simulink model "printable_simulation"  (R2024b)
settings: Solver=ode1be  StartTime=0.0  StopTime=10  FixedStep=0.001  RelTol=1e-3
model workspace (MAT data in the model file):
  AMP = 1
  FREQ = 1
  i_abc = 1
undefined symbols (not defined in the file or in its folder): Drive_wheel, Driveshaft, eff_shaft, f_OVD, i, J_S21, Jr2, K, M_curve_1, M_curve_2, M_total, mi_c, mi_s, Mode, N_clutch, n_curve_1, n_curve_2, n_max_1, n_max_2, n_surfaces, Pl, r_eq_clutch, r_geom, Shaft, sigma0, sigma1, sigma2, Spurs_Inertia, Stage1, Stage2, Stage3, vs, wheel_width
libraries: simulink x12, slpidlib x1
(part 1 of 3)
settings Model: Creator=menda  LastModifiedBy=menda
settings SolverCC: ZeroCrossAlgorithm=Adaptive
settings DebuggingCC: AlgebraicLoopMsg=none  IgnoredZcDiagnostic=none

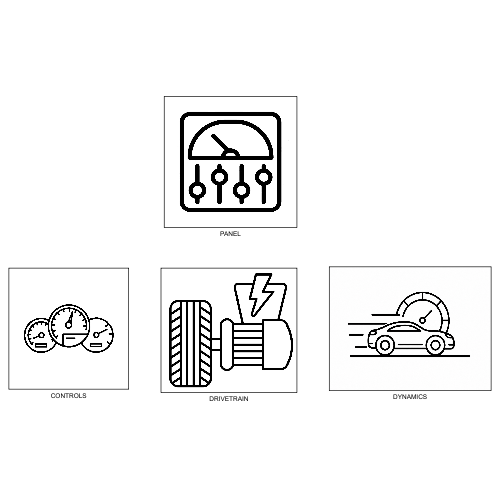
[thumbnail: Simulink's stored preview of the top-level diagram]
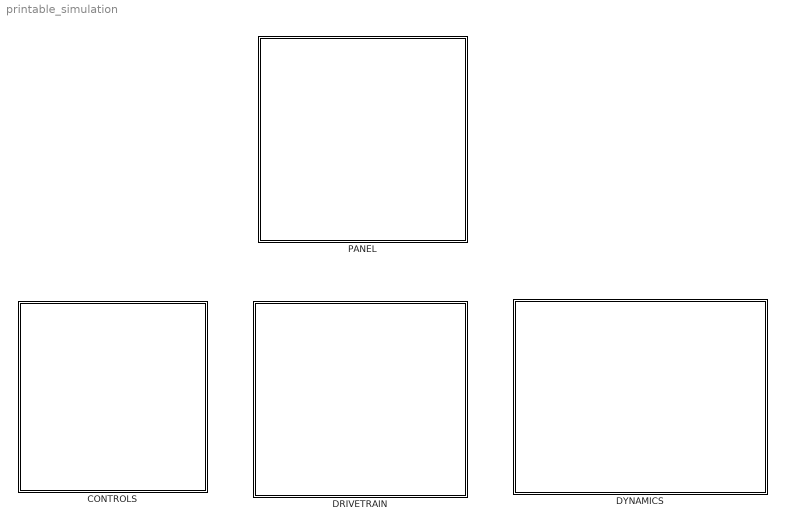
== system printable_simulation ==
  CONTROLS : Subsystem
      mask Display: image('images/controls.jpg');
  DRIVETRAIN : Subsystem
      mask Display: image('images/drivetrain_icon.png');
  DYNAMICS : Subsystem
      mask Display: image('images/Dynamics.png');
  PANEL : Subsystem
      mask Display: image('images/panel.jpg');

== system printable_simulation/CONTROLS ==
  MCU : Subsystem
      mask Display: image('images/MCU.jpg');
  Speed Profile : Subsystem
      mask Display: image('images/speedProfile.png');
  Speed control : Subsystem
      mask Display: image('images/speedControl.jpg');
  tag scope: Gear=global, M_Driver=global, M_MCU=global
  wires:
  Speed Profile/1(Target) -> Speed control/2(Target)  "v/a"
  Speed control/1(M_request) -> MCU/1(In1), [M_Driver]
  [Speed] -> Speed control/1(V_fdbk)
  MCU/1(Out1) -> [M_MCU]  "Torque"
  MCU/2(Out2) -> [Gear]  "Gear"

== system printable_simulation/DRIVETRAIN ==
  Motor : Subsystem
      mask Display: image("images/engine.jpg")
  Transmission : Subsystem
      mask Display: image('images/transmission.jpg');
  Wheel Model : Subsystem
      mask Display: image('images/wheel_model.jpg');
  Zero : Constant  Value=0  OutDataTypeStr=Inherit: Inherit via back propagation
  tag scope: F_wheel=global, M_engine=global
  wires:
  Motor/1(M_motor) -> Transmission/1(M_engine), [M_engine]
  Wheel Model/1("  ") -> [F_wheel]  "F_wheels"
  [M_MCU] -> Motor/1(M_MCU)
  Zero/1 -> Wheel Model/3(M_break)
  Transmission/1(M_tra) -> Wheel Model/2(M_tra)
  [V_load] -> Wheel Model/1(Vload)

== system printable_simulation/DYNAMICS ==
  Aerodynamic Forces : Subsystem
      mask Display: image('images/aerodynamic.png');
  Inclination : Subsystem
      mask Display: image('images/slope.jpg');
  Load Transfer : Subsystem
      mask Display: image('images/Load_transfer.png');
  Rolling Resistance : Subsystem
      mask Display: image('images/rolling_resistance.png');
  Sum : Sum  Inputs=-+-
  Vehicle Dynamics : Subsystem
      mask Display: image('images/Dynamics.png');
  tag scope: Speed=global, V_load=global
  wires:
  Sum/1 -> Vehicle Dynamics/1(Ft)
  Rolling Resistance/1(F) -> Sum/2  "F_T"
  Inclination/1(F_G) -> Sum/3  "F_G"
  Aerodynamic Forces/1(Fa) -> Sum/1  "D_A"
  Vehicle Dynamics/1(v) -> [Speed]  "v"
  [Speed] -> Rolling Resistance/1(v_x), Aerodynamic Forces/1(v_x)
  Load Transfer/1(Fz) -> [V_load]
  Vehicle Dynamics/2(acc) -> Load Transfer/1(acc)  "acc"
  Inclination/2(theta) -> Load Transfer/2(theta)  "theta"
  [F_wheel] -> Rolling Resistance/2(Fw)  "Fx"
  [V_load] -> Rolling Resistance/3(Fz)

== system printable_simulation/PANEL ==
  Differential and Driveshafts : Subsystem
      mask Display: image('images/transmission.jpg');
  Gearbox : Subsystem  Variant=on
      settings: PortSchema="{\"entries\":[{\"content\":{\"sides\":[{\"content\":{\"connectorIds\":[\"In1\"]},\"type\":\"ConnectorPlacement.EquallySpacedRectSide\",\"uuid\":\"205e71ba-e400-46cb-8798-7dc05ab83482\"},{\"content\":{\"connectorIds\":[\"Out1\"],\"side\":\"RIGHT\"},\"type\":\"ConnectorPlacement.EquallySpacedRectSide\",\"uuid\":\"765c3a3a-64c2-415f-a9cc-3b16fa892d5b\"},{\"content\":{\"connectorIds\":[\"In2\"],\"side\":\"TOP\"},\"type\":\"ConnectorPlacement.EquallySpacedRectSide\",\"uuid\":\"cfd783c5-1c77-446c-8167-ee8726316dc7\"}]},\"type\":\"ConnectorPlacement.EquallySpacedConnector\",\"uuid\":\"e0fc6072-49b0-4dfc-b677-eb2d55a08206\"}],\"packageUris\":[\"http://schema.mathworks.com/mf0/Connector/R2020b\"],\"version\":\"1.0\"}"
      mask Display: image('images/Gearbox.png');
  Main Control Unit : Subsystem
      settings: PortSchema="{\"entries\":[{\"content\":{\"sides\":[{\"content\":{\"connectorIds\":[\"In1\"]},\"type\":\"ConnectorPlacement.EquallySpacedRectSide\",\"uuid\":\"5eb0ff4b-93e1-4f3c-b7be-4fa0816a4baa\"},{\"content\":{\"side\":\"RIGHT\"},\"type\":\"ConnectorPlacement.EquallySpacedRectSide\",\"uuid\":\"5fe0ae6b-cde3-4045-ae61-047bb7dc3994\"},{\"content\":{\"side\":\"TOP\"},\"type\":\"ConnectorPlacement.EquallySpacedRectSide\",\"uuid\":\"de997b44-717c-495a-94b2-5a947ffcf83c\"},{\"content\":{\"connectorIds\":[\"Out1\",\"Out2\"],\"side\":\"BOTTOM\"},\"type\":\"ConnectorPlacement.EquallySpacedRectSide\",\"uuid\":\"4ff163e0-fe89-465b-a414-8c0cdfc889e5\"}]},\"type\":\"ConnectorPlacement.EquallySpacedConnector\",\"uuid\":\"bd974712-b545-4b72-b6b5-729f52311d40\"}],\"packageUris\":[\"http://schema.mathworks.com/mf0/Connector/R2020b\"],\"version\":\"1.0\"}"
      mask Display: image('images/MCU.jpg');
  Motor : Subsystem
      settings: PortSchema="{\"entries\":[{\"content\":{\"sides\":[{\"content\":{},\"type\":\"ConnectorPlacement.EquallySpacedRectSide\",\"uuid\":\"c3efcd4e-0739-476f-ba2f-028379b282a4\"},{\"content\":{\"connectorIds\":[\"Out1\"],\"side\":\"RIGHT\"},\"type\":\"ConnectorPlacement.EquallySpacedRectSide\",\"uuid\":\"1e8de8b1-ce2e-4e7d-9395-8c2bdb446185\"},{\"content\":{\"connectorIds\":[\"In1\"],\"side\":\"TOP\"},\"type\":\"ConnectorPlacement.EquallySpacedRectSide\",\"uuid\":\"8aefb245-65c2-4998-a20e-c273ac432bb8\"}]},\"type\":\"ConnectorPlacement.EquallySpacedConnector\",\"uuid\":\"e54aecd9-b953-4a93-9e93-d889ce431bd3\"}],\"packageUris\":[\"http://schema.mathworks.com/mf0/Connector/R2020b\"],\"version\":\"1.0\"}"
      mask Display: image("images/engine2.jpg")
  tag scope: M_tra=global
  wires:
  Motor/1(Out1) -> Gearbox/1(M_engine)  "M_motor"
  Main Control Unit/1(Out2) -> Motor/1(In1)  "M_MCU"
  Main Control Unit/2(Out1) -> Gearbox/2(Gear)  "Gear"
  Differential and Driveshafts/1(Out1) -> [M_tra]
  [M_Driver] -> Main Control Unit/1(In1)
  Gearbox/1(M_Diff) -> Differential and Driveshafts/1(In1)  "M_Diff"

== system printable_simulation/CONTROLS/MCU ==
  In1 : Inport
  clutchSet : Inport  Port=2
  AMT : Stateflow chart  Commented=on  TreatAsAtomicUnit=on
  Bus Creator : BusCreator  Inputs=2
  DCT_MCU : Stateflow chart  TreatAsAtomicUnit=on
      settings: PortSchema="{\"entries\":[{\"content\":{\"sides\":[{\"content\":{\"connectorIds\":[\"In2\",\"In1\",\"In14\",\"In9\",\"In4\",\"In5\",\"In6\",\"In16\",\"In8\",\"In15\",\"In11\",\"In12\",\"In10\",\"In13\",\"In7\",\"In3\",\"In17\"]},\"type\":\"ConnectorPlacement.EquallySpacedRectSide\",\"uuid\":\"1fb08156-1d34-4e57-90fe-6c8713929a60\"},{\"content\":{\"connectorIds\":[\"Out1\",\"Out2\",\"Out7\",\"Out4\",\"Out8\",\"Out9\",\"Out5\",\"Out6\",\"Out3\"],\"side\":\"RIGHT\"},\"type\":\"ConnectorPlacement.EquallySpacedRectSide\",\"uuid\":\"168ad19e-6ddc-4b37-b106-ff21161f873d\"},{\"content\":{\"side\":\"TOP\"},\"type\":\"ConnectorPlacement.EquallySpacedRectSide\",\"uuid\":\"0fbd732c-56c3-431e-92eb-9e0a9524aa51\"}]},\"type\":\"ConnectorPlacement.EquallySpacedConnector\",\"uuid\":\"e654060b-9493-42bd-b3b5-2b9fb4d828c1\"}],\"packageUris\":[\"http://schema.mathworks.com/mf0/Connector/R2020b\"],\"version\":\"1.0\"}"
  Gain : Gain
  Subsystem : Subsystem
  TDT : Stateflow chart  TreatAsAtomicUnit=on
  Out1 : Outport
  Out2 : Outport  Port=2
  C2 : Outport  Port=3
  tag scope: clutch=global, shifting_stage=global
  wires:
  In1/1 -> [shifting_stage], Bus Creator/1, Gain/1  "M_MCU1"
  Bus Creator/1 -> Out1/1
  Gain/1 -> Bus Creator/2  "M_MCU2"
  clutchSet/1 -> Subsystem/1(clutchSet)
  Subsystem/1(clutch) -> [clutch], C2/1

== system printable_simulation/CONTROLS/Speed Profile ==
  Acceleration Mode : Subsystem
      mask Display: image("images\AccProfile.jpg")
  Constant : Constant  Value=Mode
  Multiport Switch : MultiPortSwitch  SaturateOnIntegerOverflow=off  InputSameDT=off
  "Pedal Profile " : Subsystem
      mask Display: image("images/Pedal.jpg")
  WLTP Profile : Subsystem
      mask Display: image("images\WLTPprofile.png")
  Target : Outport
  wires:
  Multiport Switch/1 -> Target/1
  Acceleration Mode/1(Out1) -> Multiport Switch/2
  WLTP Profile/1(Out1) -> Multiport Switch/3
  "Pedal Profile "/1(Out1) -> Multiport Switch/4
  Constant/1 -> Multiport Switch/1

== system printable_simulation/CONTROLS/Speed control ==
  V_fdbk : Inport
  Target : Inport  Port=2
  Add : Sum  Inputs=+-
  Constant : Constant  Value=Mode
  Gain : Gain  Gain=3.6
  Gain1 : Gain  Gain=M_total
  Pedal Value Limiter : Saturate  UpperLimit=1  LowerLimit=-1
  Speed Control : slpidlib/PID Controller  Controller=PID  Form=Parallel  TimeDomain=Continuous-time  UseExternalTs=off  SampleTime=-1  IntegratorMethod=Forward Euler  FilterMethod=Forward Euler  ControllerParametersSource=internal  P=0.8  I=0.001  UseKiTs=off  D=0  UseExternalDerivativeSource=off  N=100  UseFilter=on  TunerSelectOption=Transfer Function Based (PID Tuner App)  InitialConditionSource=internal  InitialConditionForIntegrator=0  InitialConditionForFilter=0  DifferentiatorICPrevScaledInput=0  ExternalReset=none  TrackingMode=off  Kt=1  LimitOutput=off  SatLimitsSource=internal  UpperSaturationLimit=inf  LowerSaturationLimit=-inf  LinearizeAsGain=on  AntiWindupMode=none  Kb=1  LimitIntegrator=off  UpperIntegratorSaturationLimit=inf  LowerIntegratorSaturationLimit=-inf  POutMin=[]  POutMax=[]  IOutMin=[]  IOutMax=[]  DOutMin=[]  DOutMax=[]  NOutMin=[]  NOutMax=[]  SumOutMin=[]  SumOutMax=[]  SaturationOutMin=[]  SaturationOutMax=[]  PParamMin=[]  PParamMax=[]  IParamMin=[]  IParamMax=[]  DParamMin=[]  DParamMax=[]  NParamMin=[]  NParamMax=[]  KbParamMin=[]  KbParamMax=[]  KtParamMin=[]  KtParamMax=[]  KbOutMin=[]  KbOutMax=[]  KtOutMin=[]  KtOutMax=[]  IntegratorOutMin=[]  IntegratorOutMax=[]  FilterOutMin=[]  FilterOutMax=[]  SumI1OutMin=[]  SumI1OutMax=[]  SumI2OutMin=[]  SumI2OutMax=[]  SumI3OutMin=[]  SumI3OutMax=[]  SumI4OutMin=[]  SumI4OutMax=[]  SumDOutMin=[]  SumDOutMax=[]  DifferentiatorOutMin=[]  DifferentiatorOutMax=[]  FilterDiffOutCoefMin=[]  FilterDiffOutCoefMax=[]  ReciprocalOutMin=[]  ReciprocalOutMax=[]  SumDenOutMin=[]  SumDenOutMax=[]  SumNumOutMin=[]  SumNumOutMax=[]  DivideOutMin=[]  DivideOutMax=[]  UdiffTsProdOutMin=[]  UdiffTsProdOutMax=[]  NTsProdOutMin=[]  NTsProdOutMax=[]  UintegralTsProdOutMin=[]  UintegralTsProdOutMax=[]  UngainTsProdOutMin=[]  UngainTsProdOutMax=[]  ClampingZeroOutDataTypeStr=Inherit: Inherit via back propagation  ClampingZeroOutMin=[]  ClampingZeroOutMax=[]  FilterDenConstantOutDataTypeStr=Inherit: Inherit via back propagation  FilterDenConstantOutMin=[]  FilterDenConstantOutMax=[]  PCopyOutDataTypeStr=Inherit: Inherit via back propagation  PCopyOutMin=[]  PCopyOutMax=[]  NCopyOutDataTypeStr=Inherit: Inherit via back propagation  NCopyOutMin=[]  NCopyOutMax=[]  IntegratorContinuousStateAttributes=''  IntegratorStateMustResolveToSignalObject=off  IntegratorRTWStateStorageClass=Auto  FilterContinuousStateAttributes=''  FilterStateMustResolveToSignalObject=off  FilterRTWStateStorageClass=Auto  ParallelPVariant=InternalParameters  IdealPVariant=Disabled  IVariant=InternalParameters  DVariant=InternalParameters  IntegratorVariant=Continuous  SatVariant=Disabled  AWVariant=Passthrough  PCopyVariant=Disabled  TRVariant=Disabled  FdbkBlocksVariant=Forward  IdealPFdbkVariant=Disabled  SatFdbkVariant=Disabled  DerivativeFilterVariant=ContFilter  NVariant=InternalParameters  NCopyVariant=Disabled  FilterICVariant=InternalICsFilter  IntegratorICVariant=InternalICs  ExternalResetVariant=Disabled  TRSumVariant=Passthrough  SumFdbkVariant=Disabled  SumVariant=Sum_PID  TsampFilterVariant=InternalTs  TsampNgainVariant=Passthrough  TsampIntegralVariant=Disabled_SignalSpec  ExternalSaturationOutDataTypeStr=Inherit: Same as second input  DerivativeSourceVariant=ErrorSignal  PreIntVariant=InternalPreInt
  Switch : Switch  Criteria=u2 > Threshold  Threshold=2  SaturateOnIntegerOverflow=off  InputSameDT=off
  Transfer Fcn : TransferFcn  Denominator=[0.008 1]
  M_request : Outport
  tag scope: Pedal=global
  wires:
  Add/1 -> Speed Control/1  "v_error"
  Transfer Fcn/1 -> Gain1/1, [Pedal]  "Pedal_value"
  Constant/1 -> Switch/2
  Gain1/1 -> M_request/1
  Pedal Value Limiter/1 -> Switch/3
  Speed Control/1 -> Pedal Value Limiter/1
  Gain/1 -> Add/2
  Switch/1 -> Transfer Fcn/1
  Target/1 -> Add/1, Switch/1
  V_fdbk/1 -> Gain/1

== system printable_simulation/DRIVETRAIN/Motor ==
  M_MCU : Inport
  AND : Logic  Inputs=3  IconShape=distinctive  AllPortsSameDT=off  OutDataTypeStr=boolean
  Subsystem : Subsystem  Commented=on
  Subsystem1 : Subsystem  Commented=on
  Subsystem2 : Subsystem
  M_motor : Outport
  wires:
  M_MCU/1 -> Subsystem2/1(M_MCU), Subsystem1/1(M_MCU), Subsystem/1(M_MCU)
  Subsystem/1(M_motor) -> AND/3  "M_motor"
  AND/1 -> M_motor/1
  Subsystem1/1(M_motor) -> AND/2
  Subsystem2/1(M_motor) -> AND/1

== system printable_simulation/DRIVETRAIN/Transmission ==
  M_engine : Inport
  Differential and Driveshafts : Subsystem
      mask Display: image('images/transmission.jpg');
  Gearbox : Subsystem  Variant=on
      mask Display: image('images/branco.png');
  eff_GB : Gain  Gain=0.97
  M_tra : Outport
  wires:
  M_engine/1 -> Gearbox/1(M_motor)
  Gearbox/1(M_Diff) -> eff_GB/1
  eff_GB/1 -> Differential and Driveshafts/1(M_Diff)
  Differential and Driveshafts/1(M_shaftL) -> M_tra/1

== system printable_simulation/DRIVETRAIN/Wheel Model ==
  Vload : Inport
  M_tra : Inport  Port=2
  M_break : Inport  Port=3
  Front Wheels : Subsystem
      mask Display: image('images/branco.png');
  Product : Product
  Rear Wheels : Subsystem
      mask Display: image('images/branco.png');
  Sum : Sum  Inputs=+|+
  "  " : Outport
  tag scope: w_fdbk_tire=global
  wires:
  Sum/1 -> "  "/1
  Vload/1 -> Front Wheels/1(Vload), Rear Wheels/3(Vload)
  Rear Wheels/1(F_rear_wheels) -> Sum/1  "F_rear"
  Front Wheels/1(F_front_wheels) -> Sum/2  "F_front"
  M_tra/1 -> Rear Wheels/1(M_tra), Front Wheels/2(M_tra)
  M_break/1 -> Front Wheels/3(M_break), Rear Wheels/2(M_break)
  [Speed] -> Product/1
  [r_dyn] -> Product/2
  Product/1 -> [w_fdbk_tire]

== system printable_simulation/DYNAMICS/Aerodynamic Forces ==
  v_x : Inport
  Fa : Outport  VectorParamsAs1DForOutWhenUnconnected=off
  wires:
  v_x/1 -> Fa/1

== system printable_simulation/DYNAMICS/Inclination ==
  Constant : Constant
  Constant1 : Constant
  F_G : Outport  VectorParamsAs1DForOutWhenUnconnected=off
  theta : Outport  Port=2  VectorParamsAs1DForOutWhenUnconnected=off
  wires:
  Constant/1 -> theta/1
  Constant1/1 -> F_G/1

== system printable_simulation/DYNAMICS/Load Transfer ==
  acc : Inport
  theta : Inport  Port=2
  Terminator : Terminator
  Fz : Outport
  wires:
  acc/1 -> Fz/1
  theta/1 -> Terminator/1

== system printable_simulation/DYNAMICS/Rolling Resistance ==
  v_x : Inport
  Fw : Inport  Port=2
  Fz : Inport  Port=3
  Terminator : Terminator
  Terminator1 : Terminator
  F : Outport
  wires:
  v_x/1 -> F/1
  Fz/1 -> Terminator/1
  Fw/1 -> Terminator1/1

== system printable_simulation/DYNAMICS/Vehicle Dynamics ==
  Ft : Inport
  v : Outport
  acc : Outport  Port=2
  wires:
  Ft/1 -> acc/1, v/1  "F_tractive"

== system printable_simulation/PANEL/Differential and Driveshafts ==
  In1 : Inport
  Out1 : Outport
  wires:
  In1/1 -> Out1/1

== system printable_simulation/PANEL/Gearbox ==
  note: 1) Add Subsystem or Model blocks as valid variant choices.
      | 2) You cannot connect blocks at this level. At simulation, connectivity is automatically
      | determined, based on the active variant and port name matching.
  M_engine : Inport
  Gear : Inport  Port=2
  AMT : Subsystem  VariantControl=Gearbox == 2
      mask Display: image('images/clutch.jpg');
  AT : Subsystem  VariantControl=Gearbox == 1
      mask Display: image('images/planetary.png');
  DCT : Subsystem  VariantControl=Gearbox == 3
      mask Display: image('images/dual_clutch.png');
  TDT : Subsystem  VariantControl=Gearbox == 4
      mask Display: image('images/dog_clutch.png');
  e-CVT : Subsystem  VariantControl=Gearbox == 5
      mask Display: image('images/e-CVT.png');
  M_Diff : Outport

== system printable_simulation/PANEL/Main Control Unit ==
  In1 : Inport
  Out2 : Outport
  Out1 : Outport  Port=2
  wires:
  In1/1 -> Out1/1

== system printable_simulation/PANEL/Motor ==
  In1 : Inport
  Out1 : Outport
  wires:
  In1/1 -> Out1/1

== system printable_simulation/CONTROLS/MCU/Subsystem ==
  clutchSet : Inport
  Clock : Clock
  Delay : Delay  DelayLength=1  InitialCondition=1  InputProcessing=Columns as channels (frame based)
  Equal1 : RelationalOperator  Operator=<=  OutDataTypeStr=boolean  RndMeth=Simplest  InputSameDT=off
  Equal2 : RelationalOperator  OutDataTypeStr=boolean  RndMeth=Simplest  InputSameDT=off
  Product : Product
  Sum : Sum  Inputs=-|+
  Sum2 : Sum  Inputs=++|
  Switch : Switch  Criteria=u2 > Threshold  SaturateOnIntegerOverflow=off  InputSameDT=off
  Switch1 : Switch  Threshold=1  SaturateOnIntegerOverflow=off  InputSameDT=off
  Transport Delay : TransportDelay  DelayTime=0.001  InitialOutput=1
  signal_register : Subsystem
      mask Display: image('branco.png');
  time_register : Subsystem
  clutch : Outport
  wires:
  Delay/1 -> signal_register/1(signal), Equal2/1, Equal1/1, Switch1/1, signal_register/Trigger, time_register/Trigger
  Sum2/1 -> Equal1/2, Equal2/2, Switch1/3
  Product/1 -> Sum2/2
  signal_register/1(previous_value) -> Sum2/1
  Sum/1 -> Product/2
  Transport Delay/1 -> clutch/1
  Clock/1 -> time_register/1(t), Sum/2
  clutchSet/1 -> Delay/1
  signal_register/2(difference) -> Product/1, Switch/2
  Switch/1 -> Switch1/2
  time_register/1(t0) -> Sum/1
  Switch1/1 -> Transport Delay/1
  Equal1/1 -> Switch/1
  Equal2/1 -> Switch/3

== system printable_simulation/CONTROLS/Speed Profile/Acceleration Mode ==
  Constant : Constant
  Out1 : Outport
  wires:
  Constant/1 -> Out1/1

== system printable_simulation/CONTROLS/Speed Profile/Pedal Profile  ==
  Constant : Constant
  Out1 : Outport
  wires:
  Constant/1 -> Out1/1

== system printable_simulation/CONTROLS/Speed Profile/WLTP Profile ==
  Constant : Constant
  Out1 : Outport
  wires:
  Constant/1 -> Out1/1

== system printable_simulation/DRIVETRAIN/Motor/Subsystem ==
  M_MCU : Inport
  Compare To Constant2 : simulink/Logic and Bit Operations/Compare To Constant  relop===  const=3  OutDataTypeStr=boolean
  Engine_mech_model : Subsystem  mask{J_S1=Stage1.Spur1.J, J_S2=Stage1.Spur2.J, J_S11=Stage2.Spur11.J, J_S21=Stage2.Spur21.J, J_S12=Stage2.Spur12.J, J_S22=Stage2.Spur22.J, Jshaft=Shaft.J}
      mask prompts: J_S1 "Stage 1 Spur 1 Inertia"; J_S2 "Stage 1 Spur 2 Inertia"; J_S11 "Stage 2 Spur 11 Inertia"; J_S21 "Stage 2 Spur 21 Inertia"; J_S12 "Stage 2 Spur 12 Inertia"; J_S22 "Stage 2 Spur 22 Inertia"; Jshaft "Shaft Inertia"
      mask Display: image('images\EM_rotor.png')
  Gain2 : Gain  Gain=-1
  Integrator1 : Integrator  ExternalReset=either  InitialConditionSource=external
  "Motor_curve " : Lookup_n-D  NumberOfTableDimensions=1  BreakpointsForDimension1=n_curve_1  Table=M_curve_1  InternalRulePriority=Speed  RndMeth=Simplest
  Saturation Dynamic3 : simulink/Discontinuities/Saturation Dynamic  OutMin=[]  OutMax=[]  OutDataTypeStr=Inherit: Same as second input  OutDataType=fixdt(1, 16)  OutScaling=2^-10  DoSatur=off
  Saturation1 : Saturate  UpperLimit=n_max_1  LowerLimit=-n_max_1
  Switch1 : Switch  Criteria=u2 > Threshold  SaturateOnIntegerOverflow=off  InputSameDT=off
  Transfer Fcn4 : TransferFcn  Denominator=[0.001 1]
  "rad/s to rpm   " : Gain  Gain=60/(2*pi)
  M_motor : Outport
  tag scope: w_dot=global
  wires:
  Transfer Fcn4/1 -> M_motor/1, Engine_mech_model/1(M)  "M"
  Engine_mech_model/1(w') -> [w_dot], Integrator1/1  "w'"
  [shifting_stage] -> Compare To Constant2/1
  "rad/s to rpm   "/1 -> Saturation1/1
  Compare To Constant2/1 -> Integrator1/2, Switch1/2
  Integrator1/1 -> Switch1/1
  Switch1/1 -> "rad/s to rpm   "/1
  Gain2/1 -> Saturation Dynamic3/3
  "Motor_curve "/1 -> Gain2/1, Saturation Dynamic3/1
  Saturation1/1 -> "Motor_curve "/1  "n_motor"
  Saturation Dynamic3/1 -> Transfer Fcn4/1
  [w_motor] -> Switch1/3, Integrator1/3
  M_MCU/1 -> Saturation Dynamic3/2

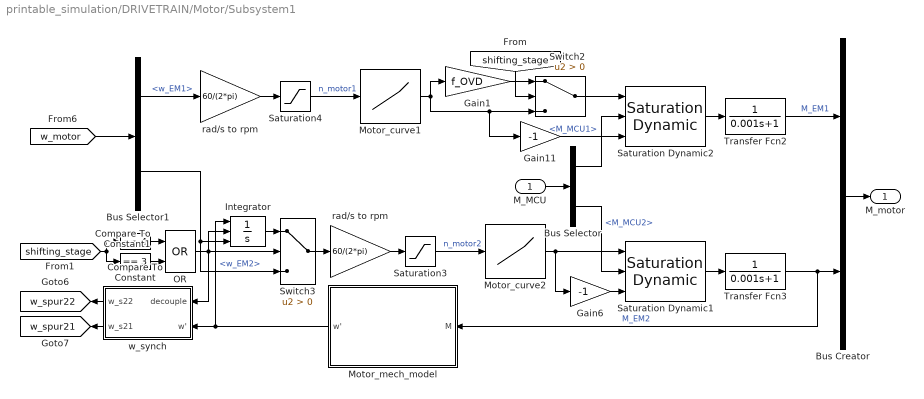
== system printable_simulation/DRIVETRAIN/Motor/Subsystem1 ==
  M_MCU : Inport
  Bus Creator : BusCreator  Inputs=2
  Bus Selector : BusSelector  OutputSignals=M_MCU1,M_MCU2
  Bus Selector1 : BusSelector  OutputSignals=w_EM1,w_EM2
  Compare To Constant : simulink/Logic and Bit Operations/Compare To Constant  relop===  const=4  OutDataTypeStr=boolean
  Compare To Constant1 : simulink/Logic and Bit Operations/Compare To Constant  relop===  const=3  OutDataTypeStr=boolean
  Gain1 : Gain  Gain=f_OVD
  Gain11 : Gain  Gain=-1
  Gain6 : Gain  Gain=-1
  Integrator : Integrator  ExternalReset=either  InitialConditionSource=external
  Motor_curve1 : Lookup_n-D  NumberOfTableDimensions=1  BreakpointsForDimension1=n_curve_1  Table=M_curve_1  InternalRulePriority=Speed  RndMeth=Simplest
  Motor_curve2 : Lookup_n-D  NumberOfTableDimensions=1  BreakpointsForDimension1=n_curve_2  Table=M_curve_2  InternalRulePriority=Speed  RndMeth=Simplest
  Motor_mech_model : Subsystem  mask{J_S1=Stage1.Spur1.J, J_S2=Stage1.Spur2.J, J_S11=Stage2.Spur11.J, J_S21=Stage2.Spur21.J, J_S12=Stage2.Spur12.J, J_S22=Stage2.Spur22.J, Jshaft=Shaft.J}
      mask prompts: J_S1 "Stage 1 Spur 1 Inertia"; J_S2 "Stage 1 Spur 2 Inertia"; J_S11 "Stage 2 Spur 11 Inertia"; J_S21 "Stage 2 Spur 21 Inertia"; J_S12 "Stage 2 Spur 12 Inertia"; J_S22 "Stage 2 Spur 22 Inertia"; Jshaft "Shaft Inertia"
      mask Display: image('images/EM_rotor.png')
  OR : Logic  Operator=OR  IconShape=distinctive  AllPortsSameDT=off  OutDataTypeStr=boolean
  Saturation Dynamic1 : simulink/Discontinuities/Saturation Dynamic  OutMin=[]  OutMax=[]  OutDataTypeStr=Inherit: Same as second input  OutDataType=fixdt(1, 16)  OutScaling=2^-10  DoSatur=off
  Saturation Dynamic2 : simulink/Discontinuities/Saturation Dynamic  OutMin=[]  OutMax=[]  OutDataTypeStr=Inherit: Same as second input  OutDataType=fixdt(1, 16)  OutScaling=2^-10  DoSatur=off
  Saturation3 : Saturate  UpperLimit=n_max_2
  Saturation4 : Saturate  UpperLimit=n_max_2
  Switch2 : Switch  Criteria=u2 > Threshold  SaturateOnIntegerOverflow=off  InputSameDT=off
  Switch3 : Switch  Criteria=u2 > Threshold  SaturateOnIntegerOverflow=off  InputSameDT=off
  Transfer Fcn2 : TransferFcn  Denominator=[0.001 1]
  Transfer Fcn3 : TransferFcn  Denominator=[0.001 1]
  "rad/s to rpm " : Gain  Gain=60/(2*pi)
  "rad/s to rpm  " : Gain  Gain=60/(2*pi)
  w_synch : Subsystem
      settings: PortSchema="{\"entries\":[{\"content\":{\"sides\":[{\"content\":{\"connectorIds\":[\"Out1\",\"Out2\"]},\"type\":\"ConnectorPlacement.EquallySpacedRectSide\",\"uuid\":\"0c74f9d6-4dd7-46ca-984a-3872ca362183\"},{\"content\":{\"connectorIds\":[\"In1\",\"In2\"],\"side\":\"RIGHT\"},\"type\":\"ConnectorPlacement.EquallySpacedRectSide\",\"uuid\":\"545eaab0-161e-407a-bd7a-8511cf00bcf5\"},{\"content\":{\"side\":\"TOP\"},\"type\":\"ConnectorPlacement.EquallySpacedRectSide\",\"uuid\":\"a44ef98a-c6fa-4a8f-9ec6-3c467f201227\"}]},\"type\":\"ConnectorPlacement.EquallySpacedConnector\",\"uuid\":\"6cdff010-dc2a-4ca6-852d-068deaf42780\"}],\"packageUris\":[\"http://schema.mathworks.com/mf0/Connector/R2020b\"],\"version\":\"1.0\"}"
      mask Display: image('images/branco.png');
  M_motor : Outport
  tag scope: w_spur21=global, w_spur22=global
  wires:
  Transfer Fcn3/1 -> Bus Creator/2, Motor_mech_model/1(M)  "M_EM2"
  Motor_curve1/1 -> Switch2/3, Gain11/1, Gain1/1
  Saturation3/1 -> Motor_curve2/1  "n_motor2"
  Bus Selector/1 -> Saturation Dynamic2/2  "<M_MCU1>"
  "rad/s to rpm "/1 -> Saturation3/1
  Compare To Constant/1 -> OR/1
  Motor_mech_model/1(w') -> w_synch/2(w'), Integrator/1
  Bus Selector1/2 -> Switch3/3, Integrator/3  "<w_EM2>"
  [shifting_stage] -> Compare To Constant1/1, Compare To Constant/1
  M_MCU/1 -> Bus Selector/1
  Motor_curve2/1 -> Saturation Dynamic1/1, Gain6/1
  Transfer Fcn2/1 -> Bus Creator/1  "M_EM1"
  w_synch/1(w_s22) -> [w_spur22]
  w_synch/2(w_s21) -> [w_spur21]
  OR/1 -> Integrator/2, w_synch/1(decouple), Switch3/2
  Gain1/1 -> Switch2/1
  [w_motor] -> Bus Selector1/1
  Integrator/1 -> Switch3/1
  Bus Selector1/1 -> "rad/s to rpm  "/1  "<w_EM1>"
  Saturation Dynamic1/1 -> Transfer Fcn3/1
  Bus Selector/2 -> Saturation Dynamic1/2  "<M_MCU2>"
  Gain6/1 -> Saturation Dynamic1/3
  Saturation Dynamic2/1 -> Transfer Fcn2/1
  "rad/s to rpm  "/1 -> Saturation4/1
  Switch2/1 -> Saturation Dynamic2/1
  Saturation4/1 -> Motor_curve1/1  "n_motor1"
  [shifting_stage] -> Switch2/2
  Compare To Constant1/1 -> OR/2
  Switch3/1 -> "rad/s to rpm "/1
  Gain11/1 -> Saturation Dynamic2/3
  Bus Creator/1 -> M_motor/1

== system printable_simulation/DRIVETRAIN/Motor/Subsystem2 ==
  M_MCU : Inport
  Gain : Gain  Gain=-1
  Motor_curve : Lookup_n-D  NumberOfTableDimensions=1  BreakpointsForDimension1=n_curve_1  Table=M_curve_1  InternalRulePriority=Speed  RndMeth=Simplest
  Saturation Dynamic : simulink/Discontinuities/Saturation Dynamic  OutMin=[]  OutMax=[]  OutDataTypeStr=Inherit: Same as second input  OutDataType=fixdt(1, 16)  OutScaling=2^-10  DoSatur=off
  Transfer Fcn1 : TransferFcn  Denominator=[0.001 1]
  max_rpm : Saturate  UpperLimit=n_max_1
  rad/s to rpm : Gain  Gain=60/(2*pi)
  M_motor : Outport
  tag scope: n_motor=global
  wires:
  Motor_curve/1 -> Gain/1, Saturation Dynamic/1
  max_rpm/1 -> Motor_curve/1, [n_motor]
  M_MCU/1 -> Saturation Dynamic/2
  [w_motor] -> rad/s to rpm/1
  Transfer Fcn1/1 -> M_motor/1
  Gain/1 -> Saturation Dynamic/3
  Saturation Dynamic/1 -> Transfer Fcn1/1
  rad/s to rpm/1 -> max_rpm/1

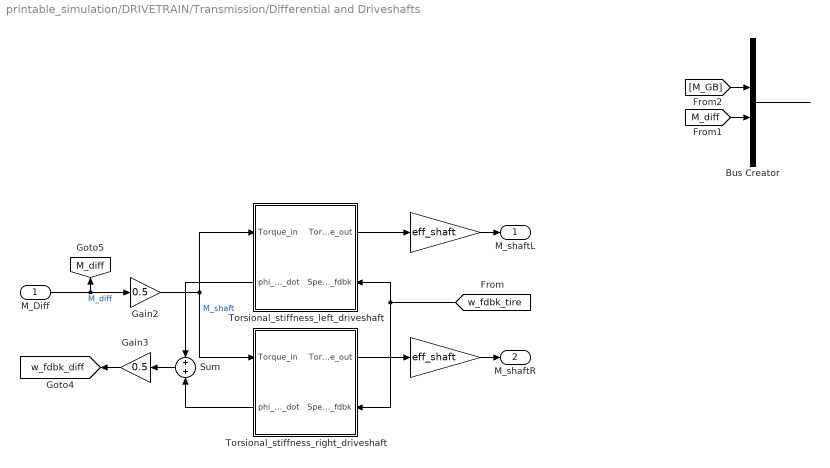
== system printable_simulation/DRIVETRAIN/Transmission/Differential and Driveshafts ==
  M_Diff : Inport
  " " : Gain  Gain=eff_shaft
  "  " : Gain  Gain=eff_shaft
  Bus Creator : BusCreator  Inputs=4
  Gain2 : Gain  Gain=0.5
  Gain3 : Gain  Gain=0.5
  Sum : Sum  Inputs=+|+
  Torsional_stiffness_left_driveshaft : Subsystem  mask{c=Driveshaft.Right.c, d=Driveshaft.Right.d, J=Driveshaft.Right.J}
      mask prompts: c "Shaft_Stiffness_Nm/rad"; d "Shaft_Damping_Nms/rad"; J "Inertia_kgm^2"
      settings: PortSchema="{\"entries\":[{\"content\":{\"sides\":[{\"content\":{\"connectorIds\":[\"In1\",\"Out2\"]},\"type\":\"ConnectorPlacement.EquallySpacedRectSide\",\"uuid\":\"898fedf9-82f7-4bc2-bf05-880de36b191d\"},{\"content\":{\"connectorIds\":[\"Out1\",\"In2\"],\"side\":\"RIGHT\"},\"type\":\"ConnectorPlacement.EquallySpacedRectSide\",\"uuid\":\"50317b6c-245f-4bd1-a8cd-7a774957ae86\"},{\"content\":{\"side\":\"TOP\"},\"type\":\"ConnectorPlacement.EquallySpacedRectSide\",\"uuid\":\"ff1de2a1-7305-40d8-9e1f-fd0fa1e7d830\"}]},\"type\":\"ConnectorPlacement.EquallySpacedConnector\",\"uuid\":\"6ce82d73-f3da-4f59-9039-464a6ef3e9c5\"}],\"packageUris\":[\"http://schema.mathworks.com/mf0/Connector/R2020b\"],\"version\":\"1.0\"}"
      mask Display: image('images/torsion.png');
  Torsional_stiffness_right_driveshaft : Subsystem  mask{c=Driveshaft.Right.c, d=Driveshaft.Right.d, J=Driveshaft.Right.J}
      mask prompts: c "Shaft_Stiffness_Nm/rad"; d "Shaft_Damping_Nms/rad"; J "Inertia_kgm^2"
      settings: PortSchema="{\"entries\":[{\"content\":{\"sides\":[{\"content\":{\"connectorIds\":[\"In1\",\"Out2\"]},\"type\":\"ConnectorPlacement.EquallySpacedRectSide\",\"uuid\":\"898fedf9-82f7-4bc2-bf05-880de36b191d\"},{\"content\":{\"connectorIds\":[\"Out1\",\"In2\"],\"side\":\"RIGHT\"},\"type\":\"ConnectorPlacement.EquallySpacedRectSide\",\"uuid\":\"50317b6c-245f-4bd1-a8cd-7a774957ae86\"},{\"content\":{\"side\":\"TOP\"},\"type\":\"ConnectorPlacement.EquallySpacedRectSide\",\"uuid\":\"ff1de2a1-7305-40d8-9e1f-fd0fa1e7d830\"}]},\"type\":\"ConnectorPlacement.EquallySpacedConnector\",\"uuid\":\"6ce82d73-f3da-4f59-9039-464a6ef3e9c5\"}],\"packageUris\":[\"http://schema.mathworks.com/mf0/Connector/R2020b\"],\"version\":\"1.0\"}"
      mask Display: image('images/torsion.png');
  M_shaftL : Outport
  M_shaftR : Outport  Port=2
  tag scope: M_diff=global, w_fdbk_diff=global
  wires:
  " "/1 -> M_shaftR/1
  "  "/1 -> M_shaftL/1
  Bus Creator/1 -> ?
  [M_diff] -> Bus Creator/3
  [M_GB] -> Bus Creator/2
  [w_fdbk_tire] -> Torsional_stiffness_right_driveshaft/2(Speed_fdbk), Torsional_stiffness_left_driveshaft/2(Speed_fdbk)
  Torsional_stiffness_right_driveshaft/1(Torque_out) -> " "/1
  Torsional_stiffness_left_driveshaft/1(Torque_out) -> "  "/1
  Sum/1 -> Gain3/1
  Gain2/1 -> Torsional_stiffness_left_driveshaft/1(Torque_in), Torsional_stiffness_right_driveshaft/1(Torque_in)  "M_shaft"
  Torsional_stiffness_left_driveshaft/2(phi_shaft_R_dot) -> Sum/1
  Gain3/1 -> [w_fdbk_diff]
  M_Diff/1 -> Gain2/1, [M_diff]  "M_diff"
  Torsional_stiffness_right_driveshaft/2(phi_shaft_R_dot) -> Sum/2

== system printable_simulation/DRIVETRAIN/Transmission/Gearbox ==
  note: 1) Add Subsystem or Model blocks as valid variant choices.
      | 2) You cannot connect blocks at this level. At simulation, connectivity is automatically
      | determined, based on the active variant and port name matching.
  M_motor : Inport
  AMT : Subsystem  VariantControl=Gearbox == 2
      mask Display: image('images/clutch.jpg');
  DCT : Subsystem  VariantControl=Gearbox == 3
      mask Display: image('images/dual_clutch.png');
  TDT : Subsystem  VariantControl=Gearbox == 4
      mask Display: image('images/dog_clutch.png');
  e-CVT : Subsystem  VariantControl=Gearbox == 5
      mask Display: image('images/e-CVT.png');
  M_Diff : Outport

== system printable_simulation/DRIVETRAIN/Wheel Model/Front Wheels ==
  Vload : Inport
  M_tra : Inport  Port=2
  M_break : Inport  Port=3
  Divide1 : Product  Inputs=/*
  Dynamic Radius : Subsystem
  Wheel Torque : Subsystem
  F_front_wheels : Outport
  wires:
  M_tra/1 -> Wheel Torque/1(M_tra)
  M_break/1 -> Wheel Torque/2(M_break)
  Wheel Torque/1(M_front_wheels) -> Divide1/2
  Vload/1 -> Dynamic Radius/1(V_load)
  Dynamic Radius/1(r_dynamic_front) -> Divide1/1
  Divide1/1 -> F_front_wheels/1

== system printable_simulation/DRIVETRAIN/Wheel Model/Rear Wheels ==
  M_tra : Inport
  M_break : Inport  Port=2
  Vload : Inport  Port=3
  Divide1 : Product  Inputs=/*
  Dynamic Radius : Subsystem
  Wheel Torque : Subsystem
  F_rear_wheels : Outport
  wires:
  Vload/1 -> Dynamic Radius/1(V_load)
  Divide1/1 -> F_rear_wheels/1
  Dynamic Radius/1(r_dynamic) -> Divide1/1
  M_tra/1 -> Wheel Torque/1(M_tra)
  M_break/1 -> Wheel Torque/2(M_break)
  Wheel Torque/1(M_rear_wheels) -> Divide1/2

== system printable_simulation/PANEL/Gearbox/AMT ==
  M_engine : Inport
  M_Diff : Outport
  wires:
  M_engine/1 -> M_Diff/1

== system printable_simulation/PANEL/Gearbox/AT ==
  M_engine : Inport
  M_Diff : Outport
  wires:
  M_engine/1 -> M_Diff/1

== system printable_simulation/PANEL/Gearbox/DCT ==
  M_engine : Inport
  M_Diff : Outport
  wires:
  M_engine/1 -> M_Diff/1

== system printable_simulation/PANEL/Gearbox/TDT ==
  M_engine : Inport
  M_Diff : Outport
  wires:
  M_engine/1 -> M_Diff/1

== system printable_simulation/PANEL/Gearbox/e-CVT ==
  M_engine : Inport
  M_Diff : Outport
  wires:
  M_engine/1 -> M_Diff/1

== system printable_simulation/CONTROLS/MCU/Subsystem/signal_register ==
  signal : Inport
  Trigger : TriggerPort  TriggerType=either  VariantControl=(inherit)  InitialTriggerSignalState=zero  PortDimensions=1
  Memory : Memory  InitialCondition=1  InheritSampleTime=on
  Subtract : Sum  Inputs=+-
  previous_value : Outport
  difference : Outport  Port=2
  wires:
  Subtract/1 -> difference/1
  Memory/1 -> Subtract/2, previous_value/1
  signal/1 -> Subtract/1, Memory/1

== system printable_simulation/CONTROLS/MCU/Subsystem/time_register ==
  t : Inport
  Trigger : TriggerPort  TriggerType=either  VariantControl=(inherit)  InitialTriggerSignalState=zero  PortDimensions=1
  t0 : Outport
  wires:
  t/1 -> t0/1

== system printable_simulation/DRIVETRAIN/Motor/Subsystem/Engine_mech_model ==
  M : Inport
  Constant : Constant  Value=Jr2+J_S1+Jshaft
  Constant2 : Constant  Value=J_S2+Jshaft+J_S11+J_S21
  Constant4 : Constant  Value=J_S22
  Constant5 : Constant  Value=J_S12
  Divide : Product  Inputs=*/
  Gain7 : Gain  Gain=1/i.S1^2
  Gain8 : Gain  Gain=1/i.S21^2
  Gain9 : Gain  Gain=1/i.S22^2
  Sum1 : Sum  Inputs=+|+
  Sum2 : Sum  Inputs=+|+
  Sum3 : Sum  Inputs=+|+
  w' : Outport
  wires:
  M/1 -> Divide/1
  Divide/1 -> w'/1
  Gain8/1 -> Sum1/2
  Gain9/1 -> Sum1/1
  Constant/1 -> Sum3/2
  Constant2/1 -> Gain7/1
  Constant4/1 -> Gain9/1
  Gain7/1 -> Sum3/1
  Sum1/1 -> Sum2/1
  Constant5/1 -> Gain8/1
  Sum3/1 -> Divide/2

== system printable_simulation/DRIVETRAIN/Motor/Subsystem1/Motor_mech_model ==
  M : Inport
  Constant : Constant  Value=Jr2+J_S1+Jshaft
  Constant2 : Constant  Value=J_S2+Jshaft+J_S11+J_S21
  Constant4 : Constant  Value=J_S22
  Constant5 : Constant  Value=J_S12
  Divide : Product  Inputs=*/
  Gain7 : Gain  Gain=1/i.S1^2
  Gain8 : Gain  Gain=1/i.S21^2
  Gain9 : Gain  Gain=1/i.S22^2
  Sum1 : Sum  Inputs=+|+
  Sum2 : Sum  Inputs=+|+
  Sum3 : Sum  Inputs=+|+
  w' : Outport
  wires:
  M/1 -> Divide/1
  Divide/1 -> w'/1
  Gain8/1 -> Sum1/2
  Gain9/1 -> Sum1/1
  Constant/1 -> Sum3/2
  Constant2/1 -> Sum2/2
  Sum2/1 -> Gain7/1
  Constant4/1 -> Gain9/1
  Gain7/1 -> Sum3/1
  Sum1/1 -> Sum2/1
  Constant5/1 -> Gain8/1
  Sum3/1 -> Divide/2

== system printable_simulation/DRIVETRAIN/Motor/Subsystem1/w_synch ==
  decouple : Inport
  w' : Inport  Port=2
  Gain2 : Gain  Gain=1/i.S22
  Gain3 : Gain  Gain=i.S21*i.S1
  Gain5 : Gain  Gain=i.S22*i.S1
  Gain7 : Gain  Gain=1/i.S21
  Integrator1 : Integrator  ExternalReset=either  InitialConditionSource=external
  Integrator2 : Integrator  ExternalReset=either  InitialConditionSource=external
  Switch4 : Switch  Criteria=u2 > Threshold  SaturateOnIntegerOverflow=off  InputSameDT=off
  Switch5 : Switch  Criteria=u2 > Threshold  SaturateOnIntegerOverflow=off  InputSameDT=off
  Switch6 : Switch  Criteria=u2 > Threshold  SaturateOnIntegerOverflow=off  InputSameDT=off
  w_s22 : Outport
  w_s21 : Outport  Port=2
  wires:
  Switch5/1 -> w_s21/1
  Integrator1/1 -> Switch4/1
  Gain3/1 -> Integrator2/1
  Switch4/1 -> w_s22/1
  decouple/1 -> Integrator1/2, Switch6/2, Switch6/3, Integrator2/2, Switch5/2, Switch4/2
  Gain5/1 -> Integrator1/1
  [w_fdbk_GB2] -> Gain2/1, Gain7/1
  Gain2/1 -> Integrator1/3, Switch4/3
  Gain7/1 -> Integrator2/3, Switch5/3
  Integrator2/1 -> Switch5/1
  w'/1 -> Switch6/1
  Switch6/1 -> Gain5/1, Gain3/1

== system printable_simulation/DRIVETRAIN/Transmission/Differential and Driveshafts/Torsional_stiffness_left_driveshaft ==
  Torque_in : Inport
  Speed_fdbk : Inport  Port=2
  Torque_out : Outport
  phi_shaft_R_dot : Outport  Port=2
  wires:
  Torque_in/1 -> phi_shaft_R_dot/1  "T_1"
  Speed_fdbk/1 -> Torque_out/1  "phi_2_dot"

== system printable_simulation/DRIVETRAIN/Transmission/Differential and Driveshafts/Torsional_stiffness_right_driveshaft ==
  Torque_in : Inport
  Speed_fdbk : Inport  Port=2
  Torque_out : Outport
  phi_shaft_R_dot : Outport  Port=2
  wires:
  Torque_in/1 -> phi_shaft_R_dot/1
  Speed_fdbk/1 -> Torque_out/1  "phi_2_dot"

== system printable_simulation/DRIVETRAIN/Transmission/Gearbox/AMT ==
  M_motor : Inport
  Clutch : Subsystem
      settings: PortSchema="{\"entries\":[{\"content\":{\"sides\":[{\"content\":{\"connectorIds\":[\"In1\",\"Out2\"]},\"type\":\"ConnectorPlacement.EquallySpacedRectSide\",\"uuid\":\"d6060937-6a70-4d8f-85b8-f3c9c5d18f93\"},{\"content\":{\"connectorIds\":[\"Out1\",\"In3\"],\"side\":\"RIGHT\"},\"type\":\"ConnectorPlacement.EquallySpacedRectSide\",\"uuid\":\"5f6b068d-fc68-4249-8013-bc3df4965ca3\"},{\"content\":{\"connectorIds\":[\"In2\"],\"side\":\"TOP\"},\"type\":\"ConnectorPlacement.EquallySpacedRectSide\",\"uuid\":\"81b536de-881e-418d-8c02-7373631e1270\"}]},\"type\":\"ConnectorPlacement.EquallySpacedConnector\",\"uuid\":\"48438dfd-c2d0-4ff7-b57e-a1bd101206eb\"}],\"packageUris\":[\"http://schema.mathworks.com/mf0/Connector/R2020b\"],\"version\":\"1.0\"}"
      mask Display: image('images/clutch.jpg');
  Multiport Switch1 : MultiPortSwitch  DataPortOrder=Zero-based contiguous  zeroidx=on  SaturateOnIntegerOverflow=off  InputSameDT=off
  Multiport Switch2 : MultiPortSwitch  DataPortOrder=Zero-based contiguous  zeroidx=on  SaturateOnIntegerOverflow=off  InputSameDT=off
  Stage1 : Subsystem  mask{i=Stage2.i1, J1=Stage2.Spur11.J, J2=Stage2.Spur12.J}
      mask prompts: i "Ratio"; J1 "Input_Gear_Inertia"; J2 "Output_Gear_Inertia"
      settings: PortSchema="{\"entries\":[{\"content\":{\"sides\":[{\"content\":{\"connectorIds\":[\"In1\",\"Out2\"]},\"type\":\"ConnectorPlacement.EquallySpacedRectSide\",\"uuid\":\"898fedf9-82f7-4bc2-bf05-880de36b191d\"},{\"content\":{\"connectorIds\":[\"Out1\",\"In2\"],\"side\":\"RIGHT\"},\"type\":\"ConnectorPlacement.EquallySpacedRectSide\",\"uuid\":\"50317b6c-245f-4bd1-a8cd-7a774957ae86\"},{\"content\":{\"side\":\"TOP\"},\"type\":\"ConnectorPlacement.EquallySpacedRectSide\",\"uuid\":\"ff1de2a1-7305-40d8-9e1f-fd0fa1e7d830\"}]},\"type\":\"ConnectorPlacement.EquallySpacedConnector\",\"uuid\":\"6ce82d73-f3da-4f59-9039-464a6ef3e9c5\"}],\"packageUris\":[\"http://schema.mathworks.com/mf0/Connector/R2020b\"],\"version\":\"1.0\"}"
      mask Display: image("images/spur_reduction.jpg");
  Stage21 : Subsystem  mask{i=Stage2.i1, J1=Stage2.Spur11.J, J2=Stage2.Spur12.J}
      mask prompts: i "Ratio"; J1 "Input_Gear_Inertia"; J2 "Output_Gear_Inertia"
      settings: PortSchema="{\"entries\":[{\"content\":{\"sides\":[{\"content\":{\"connectorIds\":[\"In1\",\"Out2\"]},\"type\":\"ConnectorPlacement.EquallySpacedRectSide\",\"uuid\":\"898fedf9-82f7-4bc2-bf05-880de36b191d\"},{\"content\":{\"connectorIds\":[\"Out1\",\"In2\"],\"side\":\"RIGHT\"},\"type\":\"ConnectorPlacement.EquallySpacedRectSide\",\"uuid\":\"50317b6c-245f-4bd1-a8cd-7a774957ae86\"},{\"content\":{\"side\":\"TOP\"},\"type\":\"ConnectorPlacement.EquallySpacedRectSide\",\"uuid\":\"ff1de2a1-7305-40d8-9e1f-fd0fa1e7d830\"}]},\"type\":\"ConnectorPlacement.EquallySpacedConnector\",\"uuid\":\"6ce82d73-f3da-4f59-9039-464a6ef3e9c5\"}],\"packageUris\":[\"http://schema.mathworks.com/mf0/Connector/R2020b\"],\"version\":\"1.0\"}"
      mask Display: image("images/spur_reduction.jpg");
  Stage22 : Subsystem  mask{i=Stage2.i1, J1=Stage2.Spur11.J, J2=Stage2.Spur12.J}
      mask prompts: i "Ratio"; J1 "Input_Gear_Inertia"; J2 "Output_Gear_Inertia"
      settings: PortSchema="{\"entries\":[{\"content\":{\"sides\":[{\"content\":{\"connectorIds\":[\"In1\",\"Out2\"]},\"type\":\"ConnectorPlacement.EquallySpacedRectSide\",\"uuid\":\"898fedf9-82f7-4bc2-bf05-880de36b191d\"},{\"content\":{\"connectorIds\":[\"Out1\",\"In2\"],\"side\":\"RIGHT\"},\"type\":\"ConnectorPlacement.EquallySpacedRectSide\",\"uuid\":\"50317b6c-245f-4bd1-a8cd-7a774957ae86\"},{\"content\":{\"side\":\"TOP\"},\"type\":\"ConnectorPlacement.EquallySpacedRectSide\",\"uuid\":\"ff1de2a1-7305-40d8-9e1f-fd0fa1e7d830\"}]},\"type\":\"ConnectorPlacement.EquallySpacedConnector\",\"uuid\":\"6ce82d73-f3da-4f59-9039-464a6ef3e9c5\"}],\"packageUris\":[\"http://schema.mathworks.com/mf0/Connector/R2020b\"],\"version\":\"1.0\"}"
      mask Display: image("images/spur_reduction.jpg");
  Stage3 : Subsystem  mask{i=Stage2.i1, J1=Stage2.Spur11.J, J2=Stage2.Spur12.J}
      mask prompts: i "Ratio"; J1 "Input_Gear_Inertia"; J2 "Output_Gear_Inertia"
      settings: PortSchema="{\"entries\":[{\"content\":{\"sides\":[{\"content\":{\"connectorIds\":[\"In1\",\"Out2\"]},\"type\":\"ConnectorPlacement.EquallySpacedRectSide\",\"uuid\":\"898fedf9-82f7-4bc2-bf05-880de36b191d\"},{\"content\":{\"connectorIds\":[\"Out1\",\"In2\"],\"side\":\"RIGHT\"},\"type\":\"ConnectorPlacement.EquallySpacedRectSide\",\"uuid\":\"50317b6c-245f-4bd1-a8cd-7a774957ae86\"},{\"content\":{\"side\":\"TOP\"},\"type\":\"ConnectorPlacement.EquallySpacedRectSide\",\"uuid\":\"ff1de2a1-7305-40d8-9e1f-fd0fa1e7d830\"}]},\"type\":\"ConnectorPlacement.EquallySpacedConnector\",\"uuid\":\"6ce82d73-f3da-4f59-9039-464a6ef3e9c5\"}],\"packageUris\":[\"http://schema.mathworks.com/mf0/Connector/R2020b\"],\"version\":\"1.0\"}"
      mask Display: image("images/spur_reduction.jpg");
  M_Diff : Outport
  tag scope: w_motor=global
  wires:
  [Gear] -> Multiport Switch1/2, Multiport Switch1/1
  Multiport Switch1/1 -> Stage3/1(Torque_in)  "M_S2"
  Stage22/1(Torque_out) -> Multiport Switch1/4
  [w_fdbk_diff] -> Stage3/2(Speed_fdbk)
  Stage22/2(phi_dot) -> Multiport Switch2/2, Multiport Switch2/4
  [Gear] -> Multiport Switch2/1
  Stage3/1(Torque_out) -> M_Diff/1
  Clutch/2(w_in) -> Stage1/2(Speed_fdbk)  "w_clutch"
  Clutch/1(M_clutch) -> Stage22/1(Torque_in), Stage21/1(Torque_in)  "M_clutch"
  Stage1/1(Torque_out) -> Clutch/1(M_in)  "M_S1"
  Stage3/2(phi_dot) -> Stage22/2(Speed_fdbk), Stage21/2(Speed_fdbk)  "w_fdbk"
  Stage1/2(phi_dot) -> [w_motor]
  M_motor/1 -> Stage1/1(Torque_in)
  [clutch] -> Clutch/2("Clutch ")
  Multiport Switch2/1 -> Clutch/3(w_out)  "w_fdbk"
  Stage21/2(phi_dot) -> Multiport Switch2/3
  Stage21/1(Torque_out) -> Multiport Switch1/3

== system printable_simulation/DRIVETRAIN/Transmission/Gearbox/DCT ==
  M_motor : Inport
  Dual_Clutch : Subsystem
      settings: PortSchema="{\"entries\":[{\"content\":{\"sides\":[{\"content\":{\"connectorIds\":[\"In1\",\"In2\",\"In3\",\"Out3\"]},\"type\":\"ConnectorPlacement.EquallySpacedRectSide\",\"uuid\":\"d6060937-6a70-4d8f-85b8-f3c9c5d18f93\"},{\"content\":{\"connectorIds\":[\"Out1\",\"In4\",\"Out2\",\"In5\"],\"side\":\"RIGHT\"},\"type\":\"ConnectorPlacement.EquallySpacedRectSide\",\"uuid\":\"5f6b068d-fc68-4249-8013-bc3df4965ca3\"},{\"content\":{\"side\":\"TOP\"},\"type\":\"ConnectorPlacement.EquallySpacedRectSide\",\"uuid\":\"81b536de-881e-418d-8c02-7373631e1270\"}]},\"type\":\"ConnectorPlacement.EquallySpacedConnector\",\"uuid\":\"48438dfd-c2d0-4ff7-b57e-a1bd101206eb\"}],\"packageUris\":[\"http://schema.mathworks.com/mf0/Connector/R2020b\"],\"version\":\"1.0\"}"
      mask Display: image('images/dual_clutch.png');
  Stage_2.1 : Subsystem  Variant=on
      settings: PortSchema="{\"entries\":[{\"content\":{\"sides\":[{\"content\":{\"connectorIds\":[\"In1\",\"Out2\"]},\"type\":\"ConnectorPlacement.EquallySpacedRectSide\",\"uuid\":\"898fedf9-82f7-4bc2-bf05-880de36b191d\"},{\"content\":{\"connectorIds\":[\"Out1\",\"In2\"],\"side\":\"RIGHT\"},\"type\":\"ConnectorPlacement.EquallySpacedRectSide\",\"uuid\":\"50317b6c-245f-4bd1-a8cd-7a774957ae86\"},{\"content\":{\"side\":\"TOP\"},\"type\":\"ConnectorPlacement.EquallySpacedRectSide\",\"uuid\":\"ff1de2a1-7305-40d8-9e1f-fd0fa1e7d830\"}]},\"type\":\"ConnectorPlacement.EquallySpacedConnector\",\"uuid\":\"6ce82d73-f3da-4f59-9039-464a6ef3e9c5\"}],\"packageUris\":[\"http://schema.mathworks.com/mf0/Connector/R2020b\"],\"version\":\"1.0\"}"
      mask Display: image('images/spur_reduction.jpg');
  Stage_2.2 : Subsystem  Variant=on
      settings: PortSchema="{\"entries\":[{\"content\":{\"sides\":[{\"content\":{\"connectorIds\":[\"In1\",\"Out2\"]},\"type\":\"ConnectorPlacement.EquallySpacedRectSide\",\"uuid\":\"898fedf9-82f7-4bc2-bf05-880de36b191d\"},{\"content\":{\"connectorIds\":[\"Out1\",\"In2\"],\"side\":\"RIGHT\"},\"type\":\"ConnectorPlacement.EquallySpacedRectSide\",\"uuid\":\"50317b6c-245f-4bd1-a8cd-7a774957ae86\"},{\"content\":{\"side\":\"TOP\"},\"type\":\"ConnectorPlacement.EquallySpacedRectSide\",\"uuid\":\"ff1de2a1-7305-40d8-9e1f-fd0fa1e7d830\"}]},\"type\":\"ConnectorPlacement.EquallySpacedConnector\",\"uuid\":\"6ce82d73-f3da-4f59-9039-464a6ef3e9c5\"}],\"packageUris\":[\"http://schema.mathworks.com/mf0/Connector/R2020b\"],\"version\":\"1.0\"}"
      mask Display: image('images/spur_reduction.jpg');
  Stage_3 : Subsystem  Variant=on
      settings: PortSchema="{\"entries\":[{\"content\":{\"sides\":[{\"content\":{\"connectorIds\":[\"In1\",\"Out2\"]},\"type\":\"ConnectorPlacement.EquallySpacedRectSide\",\"uuid\":\"37b17ee8-4b62-4191-976c-22442f171034\"},{\"content\":{\"connectorIds\":[\"Out1\",\"In2\"],\"side\":\"RIGHT\"},\"type\":\"ConnectorPlacement.EquallySpacedRectSide\",\"uuid\":\"4dd88878-371f-49ed-bf90-7ed62e5325b4\"},{\"content\":{\"side\":\"TOP\"},\"type\":\"ConnectorPlacement.EquallySpacedRectSide\",\"uuid\":\"77efb153-e78e-4021-a08b-14751aa491e1\"}]},\"type\":\"ConnectorPlacement.EquallySpacedConnector\",\"uuid\":\"fa13ac12-58ae-4dfa-a455-8cf832864b15\"}],\"packageUris\":[\"http://schema.mathworks.com/mf0/Connector/R2020b\"],\"version\":\"1.0\"}"
      mask Display: image('images/spur_reduction.jpg');
  Sum : Sum  Inputs=+|+
  M_Diff : Outport
  tag scope: w_motor=global
  wires:
  [w_fdbk_diff] -> Stage_3/2(Speed_fdbk)
  Stage_2.2/2(Speed_out) -> Dual_Clutch/5(w_out2)  "w_fdbk"
  [clutch2] -> Dual_Clutch/3(clutch2)
  Dual_Clutch/2(M_clutch2) -> Stage_2.2/1(Torque_in)  "M_clutch2"
  Stage_2.2/1(Torque_out) -> Sum/2
  Stage_3/1(Torque_out) -> M_Diff/1
  Dual_Clutch/1(M_clutch1) -> Stage_2.1/1(Torque_in)  "M_clutch1"
  Dual_Clutch/3(w_in) -> [w_motor]
  Stage_2.1/2(Speed_out) -> Dual_Clutch/4(w_out1)  "w_fdbk"
  Stage_3/2(Speed_out) -> Stage_2.1/2(Speed_fdbk), Stage_2.2/2(Speed_fdbk)  "w_fdbk"
  M_motor/1 -> Dual_Clutch/1(M_motor)
  [clutch1] -> Dual_Clutch/2(clutch1)
  Sum/1 -> Stage_3/1(Torque_in)  "M_sum"
  Stage_2.1/1(Torque_out) -> Sum/1
